simulink model "commhdlQPSKTxRxLoopback"  (R2025b)
settings: Solver=FixedStepDiscrete  StartTime=0.0  StopTime=0.03  RelTol=1e-3
PostLoadFcn:
  | hScopeConfig = get_param([gcs '/Receiver/QPSK Rx/Frequency and Time Synchronizer/Symbol Synchronizer/No HDL/QPSK Receiver Eye Diagram'],'ScopeConfiguration');
  | 
  | hScopeConfig.OpenAtSimulationStart = false;
  | hScopeConfig.Visible = false;
  | SamplesPerSymbol = 4;
  | %UpsamplesRx = 1;
  | clear hScopeConfig
InitFcn:
  | % RxAlign decoder latency (flat_simfix): 41 = netlist value used for HDL; set
  | % rxAlignLat = 25 in the base workspace before a model-level simulation.
  | if ~exist('rxAlignLat','var'), rxAlignLat = uint16(41); end
  | commhdlQPSKTxRxModelInit;
  | % Rate bridge: ADRV9002/Jupiter radio runs at 15.36 MHz = 2x the 7.68 MHz
  | % (4 samples/symbol @ Rsym=1.92 MHz) the QPSK Rx requires. The deployed
  | % Receiver must downsample the ADC stream by 2. UpsamplesRx=1 fed the QPSK
  | % Rx 8 sps (2x-upsampled) and broke symbol sync / the loopback bit check.
  | UpsamplesRx = 1;   %% T8 RATE FIX: rail 15.36e6 == ADC bus rate,
  | %% no ingress decimation (was 2 when the rail sat on the 7.68e6 rung)
  | UpsamplesTx = 1;
  | clear simTimingOffset;
StopFcn:
  | if exist('simTimingOffset','var')
  |   disp('Simulation completed');
  |   %QPSKTxRxVerification;
  | end
undefined symbols (not defined in the file or in its folder): Add, Config, fsym, randsrc, RandStream, Rsym, rxAlignLat, Shift
libraries: hdlsllib x141, simulink x45, dspsigops x30, dsphdlfiltering2 x6, dsphdlsigops2 x4, dsphdlmathfun2 x4, commdigbbndpm3 x4, dspmlti4 x2, commchan3 x1, commrflib2 x1, commcnvcod2 x1
(part 1 of 9)
CloseFcn:
  | clear Config CSLatency dataBits dataIn DBPP DescramblerLatency endLoc ...
  |         errSym errWaveform falsePacketsNo FCLatency idx initFramesNotToCompareInRx ...
  |         Nframes nReceivedBits PALatency PDLatency pktNo QPSKDemodLatency ...
  |         refQPSKSym refTxWaveform Rsym RxBits RxOut RxOutEnd RxOutSrt ...
  |         simAfterCS simBeforeSS simPeakFind simQPSKSym simSyncedPackets ...
  |         simTimingOffset simTxWaveform srtLoc SSLatency stopTime tout trueOffset ...
  |         TxBits validIn vPktNo
  | clear SamplesPerSymbol nErrBits nErrPkts nMissedPkts TxSymbolsMaxError TxWaveformMaxError
Description:
  | frame=f3072 variant=modem(sps2/Rsym7680000-T8ratefix,K5[35 23]TB25 rx+GATED-txenc,ROMf3072+byteDMA,noscr+nodescr,taps 0x150/0x154/0x15C,agcEn10,txds 0x158,WPP382) pre=variant_pre_composite_verif+cfc_a12+bytek5 build=24-Sep-2026 09:45:21 oneway=
  | 
  | FLAT REFERENCE MODEL (make_flat_model.m): every overlay applied, subsystems auto-arranged. Reading/review artefact only; the image build regenerates from commhdlQPSKTxRx.slx + the overlay stack. git=00bde48c  QPSK_LEAN=1 QPSK_FRAME=f3072 QPSK_SPS=2 QPSK_BEATFIX=1 QPSK_BEATOBS=1 QPSK_FRAMESTAT=1 QPSK_RXFIX=1 QPSK_TXFIX=1   arranged=124 skipped=89 failed=0  24-Sep-2026 09:45:31
settings Model: DataTypeOverride=Off  Creator=The MathWorks, Inc.  LastModifiedBy=tcollins
settings SolverCC: AlgebraicLoopSolver=TrustRegion  MaxZcPerStep=1.0
settings DataIOCC: ReturnWorkspaceOutputs=off
settings OptimizationCC: BlockReduction=off  ConditionallyExecuteInputs=off  DefaultParameterBehavior=Inlined  ReuseModelBlockBuffer=off
settings DebuggingCC: AlgebraicLoopMsg=error  SingleTaskRateTransMsg=error  UnconnectedInputMsg=warning  UnconnectedOutputMsg=warning  UnconnectedLineMsg=warning  SubsystemReferenceDiagnosticForUnitTest=warning
settings HardwareCC: ProdBitPerPointer=32.0  ProdBitPerSizeT=32.0  ProdBitPerPtrDiffT=32.0  ProdLargestAtomicFloat=None  ProdIntDivRoundTo=Undefined  ProdEndianess=Unspecified  ProdWordSize=32.0  ProdHWDeviceType=ASIC/FPGA->ASIC/FPGA  TargetBitPerLong=64.0  TargetBitPerPointer=64.0  TargetBitPerSizeT=64.0  TargetBitPerPtrDiffT=64.0  TargetLongLongMode=on  TargetIntDivRoundTo=Zero  TargetEndianess=LittleEndian  TargetWordSize=64.0  TargetHWDeviceType=Custom Processor->MATLAB Host Computer  ProdEqTarget=off
settings ModelReferenceCC: EnableRefExpFcnMdlSchedulingChecks=on
settings RTWCC: GPUComputeCapability=3.5  DLArmComputeVersion=19.05

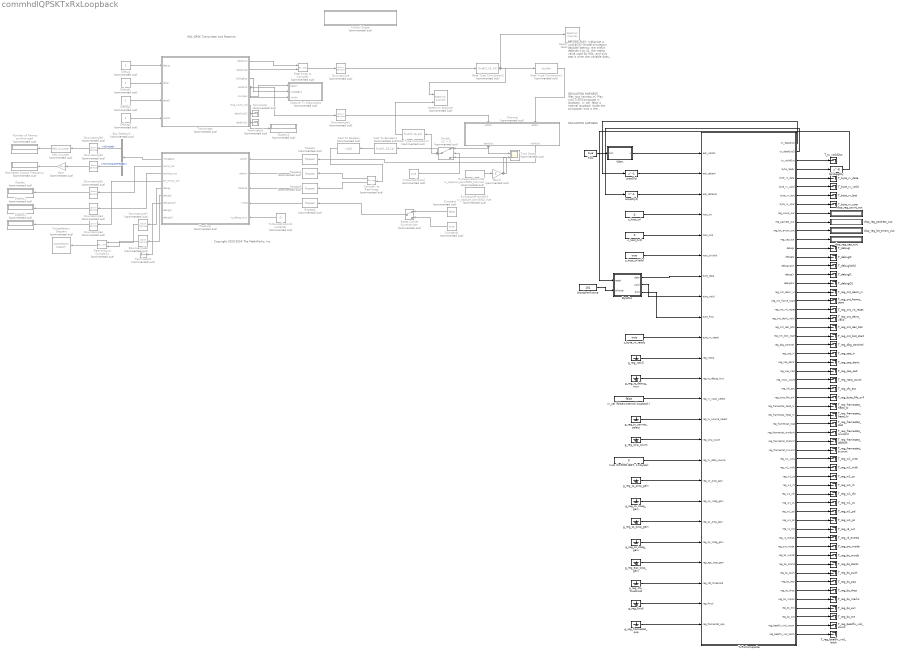
== system commhdlQPSKTxRxLoopback ==
  note: HDL QPSK Transmitter and Receiver
  note: Copyright 2020-2024 The MathWorks, Inc.
  note: SIMULATION HARNESS
  note: SIMULATION HARNESS (flat_root_harness.m)
      | Play runs TxRxComposite in loopback. rx_sel: false = internal loopback inside the composite, true = the DAC->ADC wire.
      | txds: 0 = ROM BIST frames, 1 = byte-plane source (counting words). Displays: count / packets / bit errors / cap_out (hex).
      | Logged to logsout: reg_count_out, reg_packets_out, reg_bit_errors_out, reg_cap_out, reg_cap_in, reg_cap_deint, byte_rx_data, byte_rx_valid, byte_rx_last, byte_rx_user.
      | BEFORE PLAY run   rxAlignLat = uint16(25)   in the base workspace (model sim; the InitFcn defaults it to 41, the netlist value used for HDL).
  note: BEFORE PLAY:   rxAlignLat = uint16(25)
      | (model-simulation decoder latency; the InitFcn defaults it to 41, the netlist value used for HDL,
      | and only sets it when the variable does not exist yet -- so set it yourself once per session)
  Bus Selector1 : BusSelector  Commented=on  OutputSignals=nSynced,normCoarseFreqEst
  ByteSrc : MATLAB Function  Tag=FLAT_HARNESS  TreatAsAtomicUnit=on
  Capture Tx Diagnostics : Subsystem  Commented=on
  Cast To Boolean : DataTypeConversion  Commented=on  OutDataTypeStr=int16  ConvertRealWorld=Stored Integer (SI)  SaturateOnIntegerOverflow=off  RndMeth=Floor
  Cast To Boolean1 : DataTypeConversion  Commented=on  OutDataTypeStr=fixdt(1,16,14)  SaturateOnIntegerOverflow=off  RndMeth=Floor
  Channel : Subsystem  Commented=on  mask{EbN0dB=40, CFO=1e3, CPO=135, fractionalTimingOffset=0.55, timingFrequencyOffset=2}
      mask prompts: EbN0dB "Eb/N0 (in dB) :"; CFO "Carrier Frequency Offset (in Hz):"; CPO "Carrier Phase Offset (in Degrees) :"; fractionalTimingOffset "Fractional Timing Offset ( <1 ) :"; timingFrequencyOffset "Timing Frequency Offset (in PPM) :"
      mask init:
      | validateattributes(fractionalTimingOffset,{'double'},{'finite','scalar','nonnegative','>=',0,'<',1},'','fractionalTimingOffset');
      | validateattributes(timingFrequencyOffset,{'double'},{'finite','scalar','nonnegative'},'','timingFrequencyOffset');
      | validateattributes(EbN0dB,{'double'},{'scalar'},'','EbN0dB');
      | validateattributes(CFO,{'double'},{'finite','scalar',},'','CFO');
      | validateattributes(CPO,{'double'},{'finite','scalar'},'','CPO');
      | 
      | BitsPerSymbol = 2;      % QPSK
      | EbN0          = 10^(EbN0dB/10);
      | EsN0          = BitsPerSymbol*EbN0;
      | noiseVariance = 1/EsN0;  % QPSK symbol energy is normalized to 1 i.e. Es = 1
      | 
      | clear BitsPersymbol EbN0 EsN0
      settings: PortSchema="{\"entries\":[{\"content\":{\"sides\":[{\"content\":{\"connectorIds\":[]},\"type\":\"ConnectorPlacement.EquallySpacedRectSide\",\"uuid\":\"aa9ac445-3d73-401b-8e6c-a43fa6f53e3e\"},{\"content\":{\"connectorIds\":[],\"side\":\"RIGHT\"},\"type\":\"ConnectorPlacement.EquallySpacedRectSide\",\"uuid\":\"c8fbe2c1-ad18-4b81-8824-4fece19db9b5\"},{\"content\":{\"connectorIds\":[\"In1\",\"In2\"],\"side\":\"TOP\"},\"type\":\"ConnectorPlacement.EquallySpacedRectSide\",\"uuid\":\"2fdd8701-02b7-4a19-ab6e-54d2593732fa\"},{\"content\":{\"connectorIds\":[\"Out1\",\"Out2\"],\"side\":\"BOTTOM\"},\"type\":\"ConnectorPlacement.EquallySpacedRectSide\",\"uuid\":\"bd6ca111-71ba-47de-a918-1bcd41b09175\"}]},\"type\":\"ConnectorPlacement.EquallySpacedConnector\",\"uuid\":\"c410269f-5de3-4a8f-bc07-850237ff35fb\"}],\"packageUris\":[\"http://schema.mathworks.com/mf0/Connector/R2020b\"],\"version\":\"1.0\"}"
      mask DialogControl DescGroupVar Prompt: Channel
      mask Display: disp(['Double-Click' newline 'to set channel']);
  Complex to Real-Imag : ComplexToRealImag  Commented=on
  Constant : Constant  Commented=on  Value=false  SampleTime=1/(Rsym*Config.SamplesPerSymbol)
  Constant1 : Constant  Commented=on  Value=true  SampleTime=1/(Rsym*Config.SamplesPerSymbol)
  Constellation Diagram : ConstellationDiagram  Commented=on  WindowPosition=[594.000000,164.000000,600.000000,600.000000,]  Visible=on  ScopeFrameLocation=window  SymbolsToDisplaySource=Property  SymbolsToDisplay=1000  XLimits=[-1.375,8542.5]  YLimits=[-1.375,8542.5]  AxesLimits=[-1.375,8542.5]  MaximizeAxes=on  DefaultConfigurationName=comm.scopes.ConstellationDiagramBlockCfg
  Control Scope : Subsystem  Commented=on
      settings: OpenFcn=|
      | hScopeConfig1 = get_param([gcs '/Capture Tx Diagnostics/QPSK Transmitter Constellations'],'ScopeConfiguration');
      | hScopeConfig2 = get_param([gcs '/QPSK Rx/Frequency and Time Synchronizer/Symbol Synchronizer/No HDL/QPSK Receiver Eye Diagram'],'ScopeConfiguration');
      | hScopeConfig3 = get_param([gcs '/QPSK Rx/Frequency and Time Synchronizer/Symbol Synchronizer/No HDL/No HDL/QPSK Receiver Constellation 1'],'ScopeConfiguration');
      | hScopeConfig4 = get_param([gcs '/QPSK Rx/Frequency and Time Synchronizer/No HDL/QPSK Receiver Constellations 2'],'ScopeConfiguration');
      | hScopeConfig5 = get_param([gcs '/QPSK Rx/Frequency and Time Synchronizer/Preamble Detector/No HDL/Correlation Time Scope'],'ScopeConfiguration');
      | 
      | 
      | 
      | if all([hScopeConfig1.Visible hScopeConfig2.Visible hScopeConfig3.Visible hScopeConfig4.Visible hScopeConfig5.Visible])
      |    hScopeConfig1.Visible = false;
      |    hScopeConfig2.Visible = false;
      |    hScopeConfig3.Visible = false;
      |    hScopeConfig4.Visible = false;
      |    hScopeConfig5.Visible = false;
      | else
      |    hScopeConfig1.Visible = true;
      |    hScopeConfig2.Visible = true;
      |    hScopeConfig3.Visible = true;
      |    hScopeConfig4.Visible = true;
      |    hScopeConfig5.Visible = true;
      | end
      | 
      | clear hScopeConfig1 hScopeConfig2 hScopeConfig3 hScopeConfig4 hScopeConfig5;
      mask Display: disp('Double-click to turn on/off the Scopes');
  Data Type Conversion1 : DataTypeConversion  Commented=on  OutDataTypeStr=double  SaturateOnIntegerOverflow=off  RndMeth=Floor
  Data Type Conversion2 : DataTypeConversion  Commented=on  OutDataTypeStr=fixdt(1,16,14)  ConvertRealWorld=Stored Integer (SI)  SaturateOnIntegerOverflow=off  RndMeth=Floor
  Data Type Conversion7 : DataTypeConversion  Commented=on  OutDataTypeStr=fixdt(1,16,14)  SaturateOnIntegerOverflow=off  RndMeth=Floor
  Debug : Constant  Commented=on  OutDataTypeStr=uint32  SampleTime=-1
  Debug1 : Constant  Commented=on  OutDataTypeStr=int16  SampleTime=-1
  Debug2 : Constant  Commented=on  OutDataTypeStr=int16  SampleTime=-1
  Debug3 : Constant  Commented=on  OutDataTypeStr=boolean  SampleTime=-1
  Display{,1..3} (4 alike) : Display  Commented=on
  Downsample : DownSample  Commented=on  N=UpsamplesTx  RateOptions=Allow multirate processing
  Downsample1 : DownSample  Commented=on  N=UpsamplesTx  RateOptions=Allow multirate processing
  Downsample{2..8} (7 alike) : DownSample  Commented=on  N=UpsamplesRx  RateOptions=Allow multirate processing
  Estimated Coarse Frequency : Display  Commented=on
  Gain : Gain  Commented=on  Gain=Rsym
  Gain2 : Gain  Commented=on  Gain=5
  HDL Counter : hdlsllib/Sources/HDL Counter  Commented=on  CountType=Free running  CountInit=0  CountStep=1  CountMax=25  CountFromType=Initial value  CountFrom=0  CountResetPort=off  CountLoadPort=off  CountEnbPort=on  CountDirPort=off  CountHitOutputPort=off  CountDataType=Unsigned  CountWordLen=32  CountFracLen=0  CountSampTime=1
  LoopDlyI : Delay  Tag=FLAT_HARNESS  DelayLength=1
  LoopDlyQ : Delay  Tag=FLAT_HARNESS  DelayLength=1
  Number of frames synchronized : Display  Commented=on
  Real-Imag to Complex : RealImagToComplex  Commented=on
  Real-Imag to Complex1 : RealImagToComplex  Commented=on
  Receiver : Subsystem  Commented=on  TreatAsAtomicUnit=on
  Repeat{,1..3} (4 alike) : dspsigops/Repeat  Commented=on  FactorSource=Dialog parameter  N=UpsamplesRx  Nmax=16  InputProcessing=Columns as channels (frame based)  RateOptions=Allow multirate processing  ic=0  mode=Unused parameter value
      settings: LibrarySourceBlock=commsequence2/Repeat
  Reset Carrier Synchronizer : ManualSwitch  Commented=on
  RxCaptureFromHW : FromFile  Commented=on  FileName=rx_capture_adrv9002_hdl.mat  OutDataTypeStr=double  SampleTime=1/(Rsym*Config.SamplesPerSymbol)  ExtrapolationBeforeFirstDataPoint=Hold first value  InterpolationWithinTimeRange=Zero order hold  ExtrapolationAfterLastDataPoint=Hold last value
  RxCaptureFromHW1 : FromFile  Commented=on  FileName=rx_capture_adrv9002.mat  OutDataTypeStr=double  SampleTime=1/(Rsym*Config.SamplesPerSymbol)  ExtrapolationBeforeFirstDataPoint=Hold first value  InterpolationWithinTimeRange=Zero order hold  ExtrapolationAfterLastDataPoint=Hold last value
  SkidLagDly : Delay  Tag=FLAT_HARNESS  DelayLength=8
  Spectrum Analyzer : SpectrumAnalyzer  Commented=on  NumInputPorts=2  WindowPosition=[494.000000,214.000000,800.000000,500.000000,]  Visible=on  ScopeFrameLocation=window  WindowInvariantSamplesPerUpdate=on  Span=7680000  StartFrequency=-3840000  StopFrequency=3840000  YLimits=[-47.9968 8.4452]
  Spectrum Analyzer1 : SpectrumAnalyzer  Commented=on  WindowPosition=[494.000000,214.000000,800.000000,500.000000,]  Visible=on  ScopeFrameLocation=window  WindowInvariantSamplesPerUpdate=on  Span=7680000  StartFrequency=-3840000  StopFrequency=3840000  YLimits=[-71.5508 10.9276]
  Switch : Switch  Commented=on  Criteria=u2 > Threshold  SaturateOnIntegerOverflow=off  InputSameDT=off
  T_byte_rx_data : Terminator
      settings: Tag=FLAT_HARNESS
  T_byte_rx_last : Terminator
      settings: Tag=FLAT_HARNESS
  T_byte_rx_user : Terminator
      settings: Tag=FLAT_HARNESS
  T_byte_rx_valid : Terminator
      settings: Tag=FLAT_HARNESS
  T_debugI : Terminator
      settings: Tag=FLAT_HARNESS
  T_debugI1 : Terminator
      settings: Tag=FLAT_HARNESS
  T_debugQ : Terminator
      settings: Tag=FLAT_HARNESS
  T_debugQ1 : Terminator
      settings: Tag=FLAT_HARNESS
  T_debugValid : Terminator
      settings: Tag=FLAT_HARNESS
  T_reg_beatfix_viol_count : Terminator
      settings: Tag=FLAT_HARNESS
  T_reg_beatfix_viol_latch : Terminator
      settings: Tag=FLAT_HARNESS
  T_reg_bs_cnt : Terminator
      settings: Tag=FLAT_HARNESS
  T_reg_bs_drop : Terminator
      settings: Tag=FLAT_HARNESS
  T_reg_bs_evt : Terminator
      settings: Tag=FLAT_HARNESS
  T_reg_bs_marks : Terminator
      settings: Tag=FLAT_HARNESS
  T_reg_bs_pop : Terminator
      settings: Tag=FLAT_HARNESS
  T_reg_bs_push : Terminator
      settings: Tag=FLAT_HARNESS
  T_reg_bs_starts : Terminator
      settings: Tag=FLAT_HARNESS
  T_reg_bs_words : Terminator
      settings: Tag=FLAT_HARNESS
  T_reg_byte_fifo_ovf : Terminator
      settings: Tag=FLAT_HARNESS
  T_reg_cap_cad : Terminator
      settings: Tag=FLAT_HARNESS
  T_reg_cap_deint : Terminator
      settings: Tag=FLAT_HARNESS
  T_reg_cap_in : Terminator
      settings: Tag=FLAT_HARNESS
  T_reg_cfc_est : Terminator
      settings: Tag=FLAT_HARNESS
  T_reg_cnt_bist_start : Terminator
      settings: Tag=FLAT_HARNESS
  T_reg_cnt_dec_bits : Terminator
      settings: Tag=FLAT_HARNESS
  T_reg_cnt_deint_valid : Terminator
      settings: Tag=FLAT_HARNESS
  T_reg_cnt_descr_in : Terminator
      settings: Tag=FLAT_HARNESS
  T_reg_cnt_frame_start : Terminator
      settings: Tag=FLAT_HARNESS
  T_reg_cnt_vit_reset : Terminator
      settings: Tag=FLAT_HARNESS
  T_reg_dbg_sentinel : Terminator
      settings: Tag=FLAT_HARNESS
  T_reg_framestat_head_hi : Terminator
      settings: Tag=FLAT_HARNESS
  T_reg_framestat_head_lo : Terminator
      settings: Tag=FLAT_HARNESS
  T_reg_framestat_stallcnt : Terminator
      settings: Tag=FLAT_HARNESS
  T_reg_framestat_stat : Terminator
      settings: Tag=FLAT_HARNESS
  T_reg_framestat_txurcnt : Terminator
      settings: Tag=FLAT_HARNESS
  T_reg_framestat_wordcnt : Terminator
      settings: Tag=FLAT_HARNESS
  T_reg_r4_extras : Terminator
      settings: Tag=FLAT_HARNESS
  T_reg_r4_wit : Terminator
      settings: Tag=FLAT_HARNESS
  T_reg_rstcs_count : Terminator
      settings: Tag=FLAT_HARNESS
  T_reg_sro_mode : Terminator
      settings: Tag=FLAT_HARNESS
  T_reg_w1_cfc : Terminator
      settings: Tag=FLAT_HARNESS
  T_reg_w1_cs : Terminator
      settings: Tag=FLAT_HARNESS
  T_reg_w1_pc : Terminator
      settings: Tag=FLAT_HARNESS
  T_reg_w1_pd : Terminator
      settings: Tag=FLAT_HARNESS
  T_reg_w1_rh : Terminator
      settings: Tag=FLAT_HARNESS
  T_reg_w1_ss : Terminator
      settings: Tag=FLAT_HARNESS
  T_reg_w1_wita : Terminator
      settings: Tag=FLAT_HARNESS
  T_reg_w1_witb : Terminator
      settings: Tag=FLAT_HARNESS
  T_tx_validOut : Terminator
      settings: Tag=FLAT_HARNESS
  Terminator : Terminator  Commented=on
  Terminator1 : Terminator  Commented=on
  Terminator2 : Terminator  Commented=on
  Tick : Constant  Tag=FLAT_HARNESS  Value=true  OutDataTypeStr=boolean  SampleTime=1/30.72e6
  Time Scope : Scope  Commented=on  NumInputPorts=2
      settings: TimeUnits=Metric (based on Time Span)  ActiveDisplayYMinimum=-1.0052287666621835  ActiveDisplayYMaximum=0.87958747263253323  YLabel=Amplitude
  Transmitter : Subsystem  Commented=on  TreatAsAtomicUnit=on
  TxRxComposite : Subsystem
  TxSourceControl : Constant  Commented=on  Value=true  SampleTime=-1
  TxSourceControl1 : Constant  Commented=on  Value=uint32(0)  SampleTime=-1
  VGen : MATLAB Function  Tag=FLAT_HARNESS  TreatAsAtomicUnit=on
  WordsPerFrame : Constant  Tag=FLAT_HARNESS  Value=191  OutDataTypeStr=uint32  SampleTime=1/30.72e6
  c_byte_rx_ready : Constant  Tag=FLAT_HARNESS  Value=true  OutDataTypeStr=boolean  SampleTime=1/30.72e6
  c_host_txI : Constant  Tag=FLAT_HARNESS  Value=0  OutDataTypeStr=int16  SampleTime=1/30.72e6
  c_host_txQ : Constant  Tag=FLAT_HARNESS  Value=0  OutDataTypeStr=int16  SampleTime=1/30.72e6
  c_host_txValid : Constant  Tag=FLAT_HARNESS  Value=true  OutDataTypeStr=boolean  SampleTime=1/30.72e6
  disp_reg_bit_errors_out : Display
      settings: Tag=FLAT_HARNESS
  disp_reg_cap_out : Display
      settings: Tag=FLAT_HARNESS  Format=hex (Stored Integer)
  disp_reg_count_out : Display
      settings: Tag=FLAT_HARNESS
  disp_reg_packets_out : Display
      settings: Tag=FLAT_HARNESS
  g_reg_agc_loop_gain : Ground  Tag=FLAT_HARNESS
  g_reg_cfo_threshold : Ground  Tag=FLAT_HARNESS
  g_reg_cs_integ_gain : Ground  Tag=FLAT_HARNESS
  g_reg_cs_prop_gain : Ground  Tag=FLAT_HARNESS
  g_reg_fixctl : Ground  Tag=FLAT_HARNESS
  g_reg_framestat_pop : Ground  Tag=FLAT_HARNESS
  g_reg_iq_debug_mux : Ground  Tag=FLAT_HARNESS
  g_reg_rstCS : Ground  Tag=FLAT_HARNESS
  g_reg_skip_count : Ground  Tag=FLAT_HARNESS
  g_reg_ss_integ_gain : Ground  Tag=FLAT_HARNESS
  g_reg_ss_prop_gain : Ground  Tag=FLAT_HARNESS
  g_reg_tx_source_select : Ground  Tag=FLAT_HARNESS
  rx_sel (false=internal loopback) : Constant  Tag=FLAT_HARNESS  Value=false  OutDataTypeStr=boolean  SampleTime=1/15.36e6
  "txds (0=ROM BIST, 1=bytes)" : Constant  Tag=FLAT_HARNESS  Value=0  OutDataTypeStr=uint32  SampleTime=1/15.36e6
  wires:
  TxRxComposite/57(reg_beatfix_viol_latch) -> T_reg_beatfix_viol_latch/1
  TxRxComposite/56(reg_beatfix_viol_count) -> T_reg_beatfix_viol_count/1
  TxRxComposite/55(reg_bs_cnt) -> T_reg_bs_cnt/1
  TxRxComposite/54(reg_bs_evt) -> T_reg_bs_evt/1
  TxRxComposite/53(reg_bs_marks) -> T_reg_bs_marks/1
  TxRxComposite/52(reg_bs_drop) -> T_reg_bs_drop/1
  TxRxComposite/51(reg_bs_pop) -> T_reg_bs_pop/1
  TxRxComposite/50(reg_bs_push) -> T_reg_bs_push/1
  TxRxComposite/49(reg_bs_starts) -> T_reg_bs_starts/1
  TxRxComposite/48(reg_bs_words) -> T_reg_bs_words/1
  TxRxComposite/47(reg_sro_mode) -> T_reg_sro_mode/1
  TxRxComposite/46(reg_r4_extras) -> T_reg_r4_extras/1
  TxRxComposite/45(reg_r4_wit) -> T_reg_r4_wit/1
  TxRxComposite/44(reg_w1_pc) -> T_reg_w1_pc/1
  TxRxComposite/43(reg_w1_pd) -> T_reg_w1_pd/1
  TxRxComposite/42(reg_w1_cs) -> T_reg_w1_cs/1
  TxRxComposite/41(reg_w1_cfc) -> T_reg_w1_cfc/1
  TxRxComposite/40(reg_w1_rh) -> T_reg_w1_rh/1
  TxRxComposite/39(reg_w1_ss) -> T_reg_w1_ss/1
  TxRxComposite/38(reg_w1_witb) -> T_reg_w1_witb/1
  TxRxComposite/37(reg_w1_wita) -> T_reg_w1_wita/1
  TxRxComposite/36(reg_framestat_txurcnt) -> T_reg_framestat_txurcnt/1
  TxRxComposite/35(reg_framestat_stallcnt) -> T_reg_framestat_stallcnt/1
  TxRxComposite/34(reg_framestat_wordcnt) -> T_reg_framestat_wordcnt/1
  TxRxComposite/33(reg_framestat_stat) -> T_reg_framestat_stat/1
  TxRxComposite/32(reg_framestat_head_hi) -> T_reg_framestat_head_hi/1
  TxRxComposite/31(reg_framestat_head_lo) -> T_reg_framestat_head_lo/1
  TxRxComposite/30(reg_byte_fifo_ovf) -> T_reg_byte_fifo_ovf/1
  TxRxComposite/29(reg_cfc_est) -> T_reg_cfc_est/1
  TxRxComposite/28(reg_rstcs_count) -> T_reg_rstcs_count/1
  TxRxComposite/27(reg_cap_cad) -> T_reg_cap_cad/1
  TxRxComposite/26(reg_cap_deint) -> T_reg_cap_deint/1
  TxRxComposite/25(reg_cap_in) -> T_reg_cap_in/1
  TxRxComposite/24(reg_dbg_sentinel) -> T_reg_dbg_sentinel/1
  TxRxComposite/23(reg_cnt_bist_start) -> T_reg_cnt_bist_start/1
  TxRxComposite/22(reg_cnt_dec_bits) -> T_reg_cnt_dec_bits/1
  TxRxComposite/21(reg_cnt_deint_valid) -> T_reg_cnt_deint_valid/1
  TxRxComposite/20(reg_cnt_vit_reset) -> T_reg_cnt_vit_reset/1
  TxRxComposite/19(reg_cnt_frame_start) -> T_reg_cnt_frame_start/1
  TxRxComposite/18(reg_cnt_descr_in) -> T_reg_cnt_descr_in/1
  TxRxComposite/17(debugQ1) -> T_debugQ1/1
  TxRxComposite/16(debugI1) -> T_debugI1/1
  TxRxComposite/15(debugValid) -> T_debugValid/1
  TxRxComposite/14(debugQ) -> T_debugQ/1
  TxRxComposite/13(debugI) -> T_debugI/1
  TxRxComposite/12(reg_cap_out) -> disp_reg_cap_out/1
  TxRxComposite/11(reg_bit_errors_out) -> disp_reg_bit_errors_out/1
  TxRxComposite/10(reg_packets_out) -> disp_reg_packets_out/1
  TxRxComposite/9(reg_count_out) -> disp_reg_count_out/1
  TxRxComposite/8(byte_rx_user) -> T_byte_rx_user/1
  TxRxComposite/7(byte_rx_last) -> T_byte_rx_last/1
  TxRxComposite/6(byte_rx_valid) -> T_byte_rx_valid/1
  TxRxComposite/5(byte_rx_data) -> T_byte_rx_data/1
  SkidLagDly/1 -> ByteSrc/1(ready)
  TxRxComposite/4(byte_ready) -> SkidLagDly/1
  TxRxComposite/3(tx_validOut) -> T_tx_validOut/1
  TxRxComposite/2(tx_dataOutQ) -> LoopDlyQ/1
  TxRxComposite/1(tx_dataOutI) -> LoopDlyI/1
  g_reg_framestat_pop/1 -> TxRxComposite/24(reg_framestat_pop)
  g_reg_fixctl/1 -> TxRxComposite/23(reg_fixctl)
  g_reg_cfo_threshold/1 -> TxRxComposite/22(reg_cfo_threshold)
  g_reg_agc_loop_gain/1 -> TxRxComposite/21(reg_agc_loop_gain)
  g_reg_ss_integ_gain/1 -> TxRxComposite/20(reg_ss_integ_gain)
  g_reg_ss_prop_gain/1 -> TxRxComposite/19(reg_ss_prop_gain)
  g_reg_cs_integ_gain/1 -> TxRxComposite/18(reg_cs_integ_gain)
  g_reg_cs_prop_gain/1 -> TxRxComposite/17(reg_cs_prop_gain)
  "txds (0=ROM BIST, 1=bytes)"/1 -> TxRxComposite/16(reg_tx_data_source)
  g_reg_skip_count/1 -> TxRxComposite/15(reg_skip_count)
  g_reg_tx_source_select/1 -> TxRxComposite/14(reg_tx_source_select)
  rx_sel (false=internal loopback)/1 -> TxRxComposite/13(reg_rx_input_select)
  g_reg_iq_debug_mux/1 -> TxRxComposite/12(reg_iq_debug_mux)
  g_reg_rstCS/1 -> TxRxComposite/11(reg_rstCS)
  c_byte_rx_ready/1 -> TxRxComposite/10(byte_rx_ready)
  ByteSrc/3(first) -> TxRxComposite/9(byte_first)
  ByteSrc/2(valid) -> TxRxComposite/8(byte_valid)
  ByteSrc/1(data) -> TxRxComposite/7(byte_data)
  WordsPerFrame/1 -> ByteSrc/2(nWords)
  c_host_txValid/1 -> TxRxComposite/6(host_txValid)
  c_host_txQ/1 -> TxRxComposite/5(host_txQ)
  c_host_txI/1 -> TxRxComposite/4(host_txI)
  LoopDlyQ/1 -> TxRxComposite/3(adc_dataInQ)
  LoopDlyI/1 -> TxRxComposite/2(adc_dataInI)
  VGen/1(v) -> TxRxComposite/1(adc_validIn)
  Tick/1 -> VGen/1(tick)
  Receiver/7(debugValid) -> Terminator2/1
  Real-Imag to Complex1/1 -> Constellation Diagram/1
  Downsample8/1 -> Real-Imag to Complex1/2
  Downsample7/1 -> Real-Imag to Complex1/1
  Receiver/6(debugQ) -> Downsample8/1
  Receiver/5(debugI) -> Downsample7/1
  Cast To Boolean1/1 -> Cast To Boolean/1
  Repeat3/1 -> Receiver/3(dataInQ)
  Cast To Boolean/1 -> Complex to Real-Imag/1
  Data Type Conversion7/1 -> Spectrum Analyzer/2
  Complex to Real-Imag/2 -> Repeat3/1
  Complex to Real-Imag/1 -> Repeat1/1
  TxSourceControl1/1 -> Receiver/5(iq_debug_mux)
  Transmitter/8(dataOutI2) -> Terminator1/1
  Transmitter/7(dataOutQ2) -> Terminator/1
  Downsample6/1 -> HDL Counter/1
  Downsample5/1 -> Gain/1
  Receiver/1(rxDiagBus) -> Bus Selector1/1
  Downsample4/1 -> Display2/1
  Downsample3/1 -> Display1/1
  Downsample2/1 -> Display/1
  Repeat2/1 -> Receiver/4(rstCS)
  Repeat1/1 -> Receiver/2(dataInI)
  Repeat/1 -> Receiver/1(validIn)
  Downsample1/1 -> Channel/1(validIn)
  Downsample/1 -> Data Type Conversion2/1
  Transmitter/6(msg_count_out) -> Display3/1
  Data Type Conversion2/1 -> Spectrum Analyzer/1, Spectrum Analyzer1/1, Data Type Conversion1/1
  Transmitter/5(complex) -> Capture Tx Diagnostics/1(dataIn)
  Real-Imag to Complex/1 -> Downsample/1
  Transmitter/2(dataOutQ) -> Real-Imag to Complex/2
  Transmitter/1(dataOutI) -> Real-Imag to Complex/1
  Debug3/1 -> Transmitter/4(validIn)
  Debug1/1 -> Transmitter/2(dataI)
  Debug2/1 -> Transmitter/3(dataQ)
  Receiver/4(bit_errors_out) -> Downsample4/1
  Receiver/3(packets_out) -> Downsample3/1
  Receiver/2(count_out) -> Downsample2/1
  Reset Carrier Synchronizer/1 -> Repeat2/1
  Channel/2(validOut) -> Repeat/1
  Debug/1 -> Transmitter/1(debug)
  Transmitter/3(txDiagBus) -> Capture Tx Diagnostics/2(txDiagBus)
  Transmitter/4(validOut) -> Downsample1/1, Capture Tx Diagnostics/3(validIn)
  Gain2/1 -> Switch/3, Time Scope/2
  RxCaptureFromHW/1 -> Gain2/1
  TxSourceControl/1 -> Switch/2
  Switch/1 -> Data Type Conversion7/1, Cast To Boolean1/1
  Channel/1(dataOut) -> Time Scope/1, Switch/1
  Constant1/1 -> Reset Carrier Synchronizer/2
  Constant/1 -> Reset Carrier Synchronizer/1
  Data Type Conversion1/1 -> Channel/2(dataIn)
  Gain/1 -> Estimated Coarse Frequency/1
  Bus Selector1/2 -> Downsample5/1  "<normCoarseFreqEst>"
  HDL Counter/1 -> Number of frames synchronized/1
  Bus Selector1/1 -> Downsample6/1  "<nSynced>"

== system commhdlQPSKTxRxLoopback/Capture Tx Diagnostics ==
  dataIn : Inport
  txDiagBus : Inport  Port=2
  validIn : Inport  Port=3
  Bus Selector : BusSelector  OutputSignals=QPSKConstellationPoints,QPSKConstellationValid
  Data Type Conversion : DataTypeConversion  OutDataTypeStr=double  SaturateOnIntegerOverflow=off  RndMeth=Floor
  Data Type Conversion1 : DataTypeConversion  OutDataTypeStr=double  SaturateOnIntegerOverflow=off  RndMeth=Floor
  QPSK Transmitter Constellations : ConstellationDiagram  NumInputPorts=2  WindowPosition=[708.000000,285.000000,372.000000,357.000000,]  Visible=on  ScopeFrameLocation=window  SymbolsToDisplaySource=Property  SymbolsToDisplay=10000  ReferenceConstellation="{[0.70711+0.70711i        -0.70711+0.70711i        -0.70711-0.70711i         0.70711-0.70711i],[0.70711+0.70711i        -0.70711+0.70711i        -0.70711-0.70711i         0.70711-0.70711i]}"  ReferenceMarker={''o'',''o''}  ReferenceColor={[1 0 0],[1 0 0]}  XLimits=[-0.94638 0.94638]  YLimits=[-0.94638 0.94638]  AxesLimits=[-0.94638 0.94638]  ShowLegend=on  DefaultConfigurationName=comm.scopes.ConstellationDiagramBlockCfg
      settings: OpenAtSimulationStart=off
  Subsystem : Subsystem
  Subsystem1 : Subsystem
  Unit Delay Enabled Synchronous : hdlsllib/Discrete/Unit Delay Enabled Synchronous  InitialCondition=0.0  SampleTime=-1
  Unit Delay Enabled Synchronous1 : hdlsllib/Discrete/Unit Delay Enabled Synchronous  InitialCondition=0.0  SampleTime=-1
  wires:
  txDiagBus/1 -> Bus Selector/1
  Bus Selector/1 -> Data Type Conversion/1  "<QPSKConstellationPoints>"
  Data Type Conversion/1 -> Unit Delay Enabled Synchronous/1, Subsystem/1(In1)
  dataIn/1 -> Data Type Conversion1/1
  Bus Selector/2 -> Subsystem/Enable, Unit Delay Enabled Synchronous/2  "<QPSKConstellationValid>"
  Data Type Conversion1/1 -> Unit Delay Enabled Synchronous1/1, Subsystem1/1(In1)
  validIn/1 -> Subsystem1/Enable, Unit Delay Enabled Synchronous1/2
  Unit Delay Enabled Synchronous1/1 -> QPSK Transmitter Constellations/2  "RRC Filtered Output"
  Unit Delay Enabled Synchronous/1 -> QPSK Transmitter Constellations/1  "Modulator Output"

== system commhdlQPSKTxRxLoopback/Channel ==
  validIn : Inport
  dataIn : Inport  Port=2
  AWGN Channel : commchan3/AWGN Channel  LegacyMode=on  NoiseMethod="Signal to noise ratio  (SNR)"  noiseMode=Variance from mask  EbNo=EbN0dB  EsNo=10  SNR=10  BitsPerSymbol=2  SignalPower=1  SpecifySymbolPeriod=off  SamplesPerSymbol=1  SymbolPeriod=1/fsym  VarianceSource=Parameter  Variance=noiseVariance  RandomStream=Global stream  Seed=67  SimulateUsing=Code generation
  Add : Sum  Inputs=|++
  Add1 : Sum  Inputs=++|
  Constant : Constant  Value=fractionalTimingOffset  SampleTime=-1
  Constant1 : Constant  Value=timingFrequencyOffset * 1e-6  SampleTime=-1
  Delay : Delay  DelayLength=1
  Mod 1 : Subsystem
  Phase/ Frequency Offset : commrflib2/Phase// Frequency Offset  phaseOffset=CPO  freqPort=off  freqOffset=CFO
  Variable Fractional Delay : dspsigops/Variable Fractional Delay  mode=OBSOLETE  modeActive=Linear  L=4  FarrowL=4  R=10  alpha=1  dmax=100  InputProcessing=Columns as channels (frame based)  ic=0  noDFT=off  fallbackFIR=Clip to the minimum value necessary for centered kernel  fallbackFarrow=Clip to the minimum value necessary for centered kernel  roundingMode=Zero  overflowMode=off
  dataOut : Outport
  validOut : Outport  Port=2
  wires:
  AWGN Channel/1 -> Phase/ Frequency Offset/1
  Variable Fractional Delay/1 -> AWGN Channel/1
  dataIn/1 -> Variable Fractional Delay/1
  Constant1/1 -> Add/1
  Delay/1 -> Add/2, Add1/2
  Add/1 -> Delay/1
  Add1/1 -> Mod 1/1(In1)
  Constant/1 -> Add1/1
  Mod 1/1(Out1) -> Variable Fractional Delay/2
  Phase/ Frequency Offset/1 -> dataOut/1
  validIn/1 -> validOut/1

== system commhdlQPSKTxRxLoopback/Control Scope ==

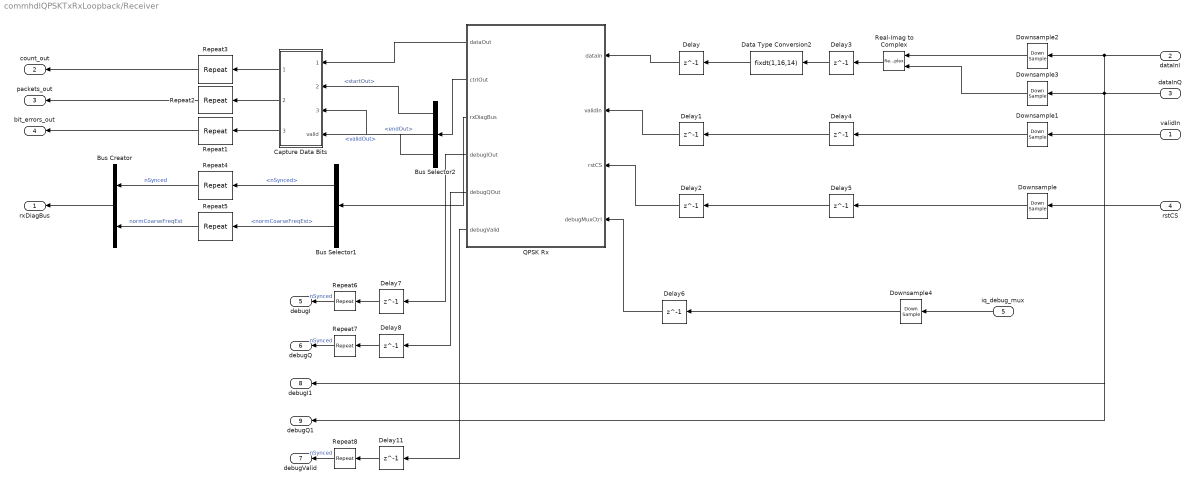
== system commhdlQPSKTxRxLoopback/Receiver ==
  validIn : Inport
  dataInI : Inport  Port=2
  dataInQ : Inport  Port=3
  rstCS : Inport  Port=4
  iq_debug_mux : Inport  Port=5  OutDataTypeStr=uint32
  Bus Creator : BusCreator  Inputs=2
  Bus Selector1 : BusSelector  OutputSignals=nSynced,normCoarseFreqEst
  Bus Selector2 : BusSelector  OutputSignals=startOut,endOut,validOut
  Capture Data Bits : Subsystem
  Data Type Conversion2 : DataTypeConversion  OutDataTypeStr=fixdt(1,16,14)  ConvertRealWorld=Stored Integer (SI)  SaturateOnIntegerOverflow=off  RndMeth=Floor
  Delay{,1..8,11} (10 alike) : Delay  DelayLength=1
  Downsample{,1..4} (5 alike) : DownSample  N=UpsamplesRx  RateOptions=Allow multirate processing
  QPSK Rx : Subsystem
      mask init:
      | integAvgLen = 2^12;
      | 
      | RxParams            = commhdlQPSKTxRxParameters();
      | Preamble            = RxParams.Preamble;
      | QPSKConstellation   = RxParams.QPSKConstellation;
      | dataBitsPerPacket   = RxParams.DataBitsPerPacket;
      | SamplesPerSymbol    = RxParams.SamplesPerSymbol;
      | RRCCoef             = RxParams.RRCCoef;
      | bitsPerPacket        = RxParams.BitsPerPacket;
      | 
      | rxPreambleMFCoeffs  = RxParams.rxPreambleMFCoeffs;
      | preambleSymbols     = RxParams.preambleSymbols;
      | ThresoldGainFac     = RxParams.ThresoldGainFac;
      | 
      | % AGC Parameters
      | AGCReference           = RxParams.AGCReference;
      | AGCLoopGain            = RxParams.AGCLoopGain;
      | 
      | % CS parameters
      | CSKp                   = RxParams.CSKp;
      | CSK0                   = RxParams.CSK0;  
      | CSLoopFilterPropGain   = RxParams.CSLoopFilterPropGain;
      | CSLoopFilterIntegGain  = RxParams.CSLoopFilterIntegGain;
      | CFOChangeDetectThreshold = RxParams.CFOChangeDetectThreshold;
      | 
      | % SS parameters
      | SSKp                   = RxParams.SSKp; 
      | SSK0                   = RxParams.SSK0;  
      | SSLoopFilterPropGain   = RxParams.SSLoopFilterPropGain;
      | SSLoopFilterIntegGain  = RxParams.SSLoopFilterIntegGain;
      | 
      | % preamble detector parameters
      | searchSamples          = RxParams.SearchSamples;
      | 
      | clear RxParams;
  Real-Imag to Complex : RealImagToComplex
  Repeat{1..8} (8 alike) : dspsigops/Repeat  FactorSource=Dialog parameter  N=UpsamplesRx  Nmax=16  InputProcessing=Columns as channels (frame based)  RateOptions=Allow multirate processing  ic=0  mode=Unused parameter value
      settings: LibrarySourceBlock=commsequence2/Repeat
  rxDiagBus : Outport
  count_out : Outport  Port=2
  packets_out : Outport  Port=3
  bit_errors_out : Outport  Port=4
  debugI : Outport  Port=5
  debugQ : Outport  Port=6
  debugValid : Outport  Port=7
  debugI1 : Outport  Port=8
  debugQ1 : Outport  Port=9
  wires:
  Bus Selector2/1 -> Capture Data Bits/2(dataSrt)  "<startOut>"
  QPSK Rx/1(dataOut) -> Capture Data Bits/1(dataOut)
  QPSK Rx/2(ctrlOut) -> Bus Selector2/1
  Bus Selector2/2 -> Capture Data Bits/3(dataEnd)  "<endOut>"
  rstCS/1 -> Downsample/1
  validIn/1 -> Downsample1/1
  Bus Selector2/3 -> Capture Data Bits/4(valid)  "<validOut>"
  Capture Data Bits/1(count_out) -> Repeat3/1
  Capture Data Bits/2(packets_out) -> Repeat2/1
  Capture Data Bits/3(bit_errors_out) -> Repeat1/1
  Downsample1/1 -> Delay4/1
  Repeat1/1 -> bit_errors_out/1
  Repeat2/1 -> packets_out/1
  Repeat3/1 -> count_out/1
  QPSK Rx/3(rxDiagBus) -> Bus Selector1/1
  Bus Creator/1 -> rxDiagBus/1
  Bus Selector1/1 -> Repeat4/1  "<nSynced>"
  Bus Selector1/2 -> Repeat5/1  "<normCoarseFreqEst>"
  Repeat4/1 -> Bus Creator/1  "nSynced"
  Repeat5/1 -> Bus Creator/2  "normCoarseFreqEst"
  dataInQ/1 -> debugQ1/1, Downsample3/1
  dataInI/1 -> debugI1/1, Downsample2/1
  Real-Imag to Complex/1 -> Delay3/1
  Downsample2/1 -> Real-Imag to Complex/1
  Downsample3/1 -> Real-Imag to Complex/2
  Data Type Conversion2/1 -> Delay/1
  Delay/1 -> QPSK Rx/1(dataIn)
  Delay1/1 -> QPSK Rx/2(validIn)
  Delay2/1 -> QPSK Rx/3(rstCS)
  Delay3/1 -> Data Type Conversion2/1
  Delay4/1 -> Delay1/1
  Delay5/1 -> Delay2/1
  QPSK Rx/4(debugIOut) -> Delay7/1
  QPSK Rx/5(debugQOut) -> Delay8/1
  Repeat6/1 -> debugI/1  "nSynced"
  Repeat7/1 -> debugQ/1  "nSynced"
  iq_debug_mux/1 -> Downsample4/1
  Delay6/1 -> QPSK Rx/4(debugMuxCtrl)
  Downsample4/1 -> Delay6/1
  Repeat8/1 -> debugValid/1  "nSynced"
  QPSK Rx/6(debugValid) -> Delay11/1
  Delay7/1 -> Repeat6/1
  Delay8/1 -> Repeat7/1
  Delay11/1 -> Repeat8/1
  Downsample/1 -> Delay5/1

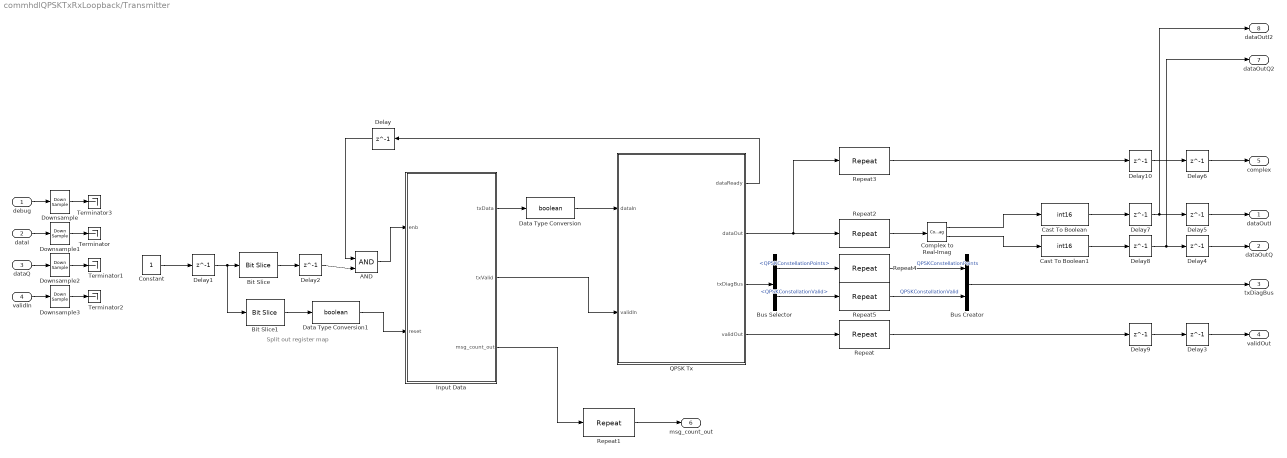
== system commhdlQPSKTxRxLoopback/Transmitter ==
  note: Split out register map
  debug : Inport  PortDimensions=1
  dataI : Inport  Port=2
  dataQ : Inport  Port=3
  validIn : Inport  Port=4
  AND : Logic  IconShape=distinctive  AllPortsSameDT=off  OutDataTypeStr=boolean
  Bit Slice : hdlsllib/Logic and Bit Operations/Bit Slice  lidx=0  ridx=0
  Bit Slice1 : hdlsllib/Logic and Bit Operations/Bit Slice  lidx=1  ridx=1
  Bus Creator : BusCreator  Inputs=2
  Bus Selector : BusSelector  OutputSignals=QPSKConstellationPoints,QPSKConstellationValid
  Cast To Boolean : DataTypeConversion  OutDataTypeStr=int16  ConvertRealWorld=Stored Integer (SI)  SaturateOnIntegerOverflow=off  RndMeth=Floor
  Cast To Boolean1 : DataTypeConversion  OutDataTypeStr=int16  ConvertRealWorld=Stored Integer (SI)  SaturateOnIntegerOverflow=off  RndMeth=Floor
  Complex to Real-Imag : ComplexToRealImag
  Constant : Constant  OutDataTypeStr=uint32  SampleTime=-1
  Data Type Conversion : DataTypeConversion  OutDataTypeStr=boolean  SaturateOnIntegerOverflow=off  RndMeth=Floor
  Data Type Conversion1 : DataTypeConversion  OutDataTypeStr=boolean  SaturateOnIntegerOverflow=off  RndMeth=Floor
  Delay{,1..10} (11 alike) : Delay  DelayLength=1
  Downsample{,1..3} (4 alike) : DownSample  N=UpsamplesTx  RateOptions=Allow multirate processing
  Input Data : Subsystem  mask{dataBits=reshape(repmat(randsrc(2240*1,1,[0,1],RandStream('mcg16807','Seed',0)), 59,1), [2240*59,1]), Rsym=7.68e6}
      mask prompts: dataBits "Data Bits :"; Rsym "Symbol Rate (in baud rate)  :"
      mask Display: disp(['Double-Click' newline 'to set data bits']);
  QPSK Tx : Subsystem
      mask init:
      | TxParams           = commhdlQPSKTxRxParameters();
      | Preamble            = TxParams.Preamble;
      | QPSKConstellation   = TxParams.QPSKConstellation;
      | dataBitsPerPacket   = TxParams.DataBitsPerPacket;
      | SamplesPerSymbol    = TxParams.SamplesPerSymbol;
      | RRCCoef             = TxParams.RRCCoef;
      | dataRAMAddrWidth    = TxParams.txDataRAMAddrWidth;
      | bitsPerPacket       = TxParams.BitsPerPacket;
      | 
      | clear TxParams;
  Repeat{,1..5} (6 alike) : dspsigops/Repeat  FactorSource=Dialog parameter  N=UpsamplesTx  Nmax=16  InputProcessing=Columns as channels (frame based)  RateOptions=Allow multirate processing  ic=0  mode=Unused parameter value
      settings: LibrarySourceBlock=commsequence2/Repeat
  Terminator{,1..3} (4 alike) : Terminator
  dataOutI : Outport
  dataOutQ : Outport  Port=2
  txDiagBus : Outport  Port=3
  validOut : Outport  Port=4
  complex : Outport  Port=5
  msg_count_out : Outport  Port=6
  dataOutQ2 : Outport  Port=7
  dataOutI2 : Outport  Port=8
  wires:
  Input Data/2(txValid) -> QPSK Tx/2(validIn)
  Input Data/1(txData) -> Data Type Conversion/1
  Data Type Conversion/1 -> QPSK Tx/1(dataIn)
  QPSK Tx/4(validOut) -> Repeat/1
  QPSK Tx/1(dataReady) -> Delay/1
  AND/1 -> Input Data/1(enb)
  Bit Slice/1 -> Delay2/1
  Delay/1 -> AND/1
  Delay1/1 -> Bit Slice1/1, Bit Slice/1
  Delay2/1 -> AND/2
  Bit Slice1/1 -> Data Type Conversion1/1
  Data Type Conversion1/1 -> Input Data/2(reset)
  dataI/1 -> Downsample1/1
  dataQ/1 -> Downsample2/1
  validIn/1 -> Downsample3/1
  Constant/1 -> Delay1/1
  debug/1 -> Downsample/1
  QPSK Tx/2(dataOut) -> Repeat3/1, Repeat2/1
  Complex to Real-Imag/1 -> Cast To Boolean/1
  Complex to Real-Imag/2 -> Cast To Boolean1/1
  Input Data/3(msg_count_out) -> Repeat1/1
  Repeat/1 -> Delay9/1
  Repeat2/1 -> Complex to Real-Imag/1
  Repeat3/1 -> Delay10/1
  Downsample/1 -> Terminator3/1
  Downsample1/1 -> Terminator/1
  Downsample2/1 -> Terminator1/1
  Downsample3/1 -> Terminator2/1
  Repeat1/1 -> msg_count_out/1
  QPSK Tx/3(txDiagBus) -> Bus Selector/1
  Bus Selector/1 -> Repeat4/1  "<QPSKConstellationPoints>"
  Repeat4/1 -> Bus Creator/1  "QPSKConstellationPoints"
  Bus Selector/2 -> Repeat5/1  "<QPSKConstellationValid>"
  Repeat5/1 -> Bus Creator/2  "QPSKConstellationValid"
  Bus Creator/1 -> txDiagBus/1
  Cast To Boolean/1 -> Delay7/1
  Cast To Boolean1/1 -> Delay8/1
  Delay3/1 -> validOut/1
  Delay4/1 -> dataOutQ/1
  Delay5/1 -> dataOutI/1
  Delay6/1 -> complex/1
  Delay7/1 -> dataOutI2/1, Delay5/1
  Delay8/1 -> dataOutQ2/1, Delay4/1
  Delay9/1 -> Delay3/1
  Delay10/1 -> Delay6/1
